simulink model "lab2"  (R2012b)
settings: Solver=ode45  StartTime=0.0  StopTime=10.0  RelTol=1e-3
undefined symbols (not defined in the file): des, gcbh
settings Model: Creator=Student  LastModifiedBy=Student

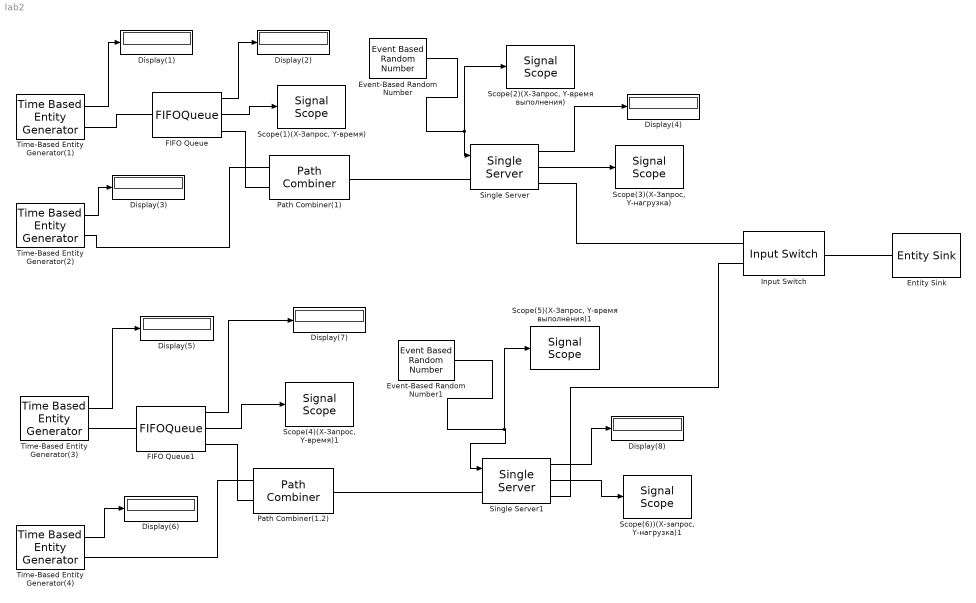
== system lab2 ==
  "Display(1) " : Display
  "Display(2) " : Display
  Display(3) : Display
  Display(4) : Display
  Display(5) : Display
  Display(6) : Display
  Display(7) : Display
  Display(8) : Display
  Entity Sink : EntitySink
  Event-Based Random Number : EventBasedRandomNumber
  Event-Based Random Number1 : EventBasedRandomNumber  meanExp=2
  FIFO Queue : FIFOQueue  StatNumberDeparted=on  StatAverageWait=on
      settings: OutputPortMap=o0,o2
  FIFO Queue1 : FIFOQueue  Capacity=30  StatNumberDeparted=on  StatAverageWait=on
      settings: OutputPortMap=o0,o2
  Input Switch : InputSwitch  NumberInputPorts=2
  Path Combiner(1) : PathCombiner  NumberInputPorts=2
  Path Combiner(1.2) : PathCombiner  NumberInputPorts=2
  "Scope(1)(X-Запрос, Y-время)" : SignalScope  LoadFcn=des.scope.CallbackSupport('seLoadFcn',gcbh)  StartFcn=des.scope.CallbackSupport('seStartFcn',gcbh)  StopFcn=des.scope.CallbackSupport('seStopFcn',gcbh)
      settings: CopyFcn=des.scope.CallbackSupport('seCopyFcn',gcbh)  DeleteFcn=des.scope.CallbackSupport('seDeleteFcn',gcbh)  PreSaveFcn=des.scope.CallbackSupport('sePreSaveFcn',gcbh)  NameChangeFcn=des.scope.CallbackSupport('seNameChangeFcn',gcbh)  OpenFcn=des.scope.CallbackSupport('seOpenFcn',gcbh)
  "Scope(2)(X-Запрос, Y-время выполнения)" : SignalScope  LoadFcn=des.scope.CallbackSupport('seLoadFcn',gcbh)  StartFcn=des.scope.CallbackSupport('seStartFcn',gcbh)  StopFcn=des.scope.CallbackSupport('seStopFcn',gcbh)
      settings: CopyFcn=des.scope.CallbackSupport('seCopyFcn',gcbh)  DeleteFcn=des.scope.CallbackSupport('seDeleteFcn',gcbh)  PreSaveFcn=des.scope.CallbackSupport('sePreSaveFcn',gcbh)  NameChangeFcn=des.scope.CallbackSupport('seNameChangeFcn',gcbh)  OpenFcn=des.scope.CallbackSupport('seOpenFcn',gcbh)
  "Scope(3)(X-Запрос, Y-нагрузка)" : SignalScope  LoadFcn=des.scope.CallbackSupport('seLoadFcn',gcbh)  StartFcn=des.scope.CallbackSupport('seStartFcn',gcbh)  StopFcn=des.scope.CallbackSupport('seStopFcn',gcbh)
      settings: CopyFcn=des.scope.CallbackSupport('seCopyFcn',gcbh)  DeleteFcn=des.scope.CallbackSupport('seDeleteFcn',gcbh)  PreSaveFcn=des.scope.CallbackSupport('sePreSaveFcn',gcbh)  NameChangeFcn=des.scope.CallbackSupport('seNameChangeFcn',gcbh)  OpenFcn=des.scope.CallbackSupport('seOpenFcn',gcbh)
  "Scope(4)(X-Запрос, Y-время)1" : SignalScope  LoadFcn=des.scope.CallbackSupport('seLoadFcn',gcbh)  StartFcn=des.scope.CallbackSupport('seStartFcn',gcbh)  StopFcn=des.scope.CallbackSupport('seStopFcn',gcbh)
      settings: CopyFcn=des.scope.CallbackSupport('seCopyFcn',gcbh)  DeleteFcn=des.scope.CallbackSupport('seDeleteFcn',gcbh)  PreSaveFcn=des.scope.CallbackSupport('sePreSaveFcn',gcbh)  NameChangeFcn=des.scope.CallbackSupport('seNameChangeFcn',gcbh)  OpenFcn=des.scope.CallbackSupport('seOpenFcn',gcbh)
  "Scope(5)(X-Запрос, Y-время выполнения)1" : SignalScope  LoadFcn=des.scope.CallbackSupport('seLoadFcn',gcbh)  StartFcn=des.scope.CallbackSupport('seStartFcn',gcbh)  StopFcn=des.scope.CallbackSupport('seStopFcn',gcbh)
      settings: CopyFcn=des.scope.CallbackSupport('seCopyFcn',gcbh)  DeleteFcn=des.scope.CallbackSupport('seDeleteFcn',gcbh)  PreSaveFcn=des.scope.CallbackSupport('sePreSaveFcn',gcbh)  NameChangeFcn=des.scope.CallbackSupport('seNameChangeFcn',gcbh)  OpenFcn=des.scope.CallbackSupport('seOpenFcn',gcbh)
  "Scope(6))(X-запрос, Y-нагрузка)1" : SignalScope  LoadFcn=des.scope.CallbackSupport('seLoadFcn',gcbh)  StartFcn=des.scope.CallbackSupport('seStartFcn',gcbh)  StopFcn=des.scope.CallbackSupport('seStopFcn',gcbh)
      settings: CopyFcn=des.scope.CallbackSupport('seCopyFcn',gcbh)  DeleteFcn=des.scope.CallbackSupport('seDeleteFcn',gcbh)  PreSaveFcn=des.scope.CallbackSupport('sePreSaveFcn',gcbh)  NameChangeFcn=des.scope.CallbackSupport('seNameChangeFcn',gcbh)  OpenFcn=des.scope.CallbackSupport('seOpenFcn',gcbh)
  Single Server : SingleServer  ServiceTimeFrom=Signal port t  PriorityServiceCompletion=50  StatNumberDeparted=on  StatUtilization=on
      settings: OutputPortMap=o0,o5
  Single Server1 : SingleServer  ServiceTimeFrom=Signal port t  PriorityServiceCompletion=50  StatNumberDeparted=on  StatUtilization=on
      settings: OutputPortMap=o0,o5
  "Time-Based Entity Generator(1) " : TimeBasedEntityGenerator  Period=3  StatNumberDeparted=on
  "Time-Based Entity Generator(2) " : TimeBasedEntityGenerator  Period=3  StatNumberDeparted=on
  Time-Based Entity Generator(3) : TimeBasedEntityGenerator  StatNumberDeparted=on
  Time-Based Entity Generator(4) : TimeBasedEntityGenerator  Period=2  StatNumberDeparted=on
  wires:
  "Time-Based Entity Generator(1) "/1 -> "Display(1) "/1
  FIFO Queue/1 -> "Display(2) "/1
  FIFO Queue/2 -> "Scope(1)(X-Запрос, Y-время)"/1
  "Time-Based Entity Generator(2) "/1 -> Display(3)/1
  Event-Based Random Number/1 -> "Scope(2)(X-Запрос, Y-время выполнения)"/1, Single Server/1
  Single Server/1 -> Display(4)/1
  Single Server/2 -> "Scope(3)(X-Запрос, Y-нагрузка)"/1
  Time-Based Entity Generator(3)/1 -> Display(5)/1
  FIFO Queue1/1 -> Display(7)/1
  FIFO Queue1/2 -> "Scope(4)(X-Запрос, Y-время)1"/1
  Time-Based Entity Generator(4)/1 -> Display(6)/1
  Event-Based Random Number1/1 -> "Scope(5)(X-Запрос, Y-время выполнения)1"/1, Single Server1/1
  Single Server1/1 -> Display(8)/1
  Single Server1/2 -> "Scope(6))(X-запрос, Y-нагрузка)1"/1
  connections:
  "Time-Based Entity Generator(1) "/RConn1 -- FIFO Queue/LConn1
  FIFO Queue/RConn1 -- Path Combiner(1)/LConn2
  "Time-Based Entity Generator(2) "/RConn1 -- Path Combiner(1)/LConn1
  Path Combiner(1)/RConn1 -- Single Server/LConn1
  Single Server/RConn1 -- Input Switch/LConn1
  Input Switch/RConn1 -- Entity Sink/LConn1
  Time-Based Entity Generator(3)/RConn1 -- FIFO Queue1/LConn1
  FIFO Queue1/RConn1 -- Path Combiner(1.2)/LConn2
  Time-Based Entity Generator(4)/RConn1 -- Path Combiner(1.2)/LConn1
  Path Combiner(1.2)/RConn1 -- Single Server1/LConn1
  Single Server1/RConn1 -- Input Switch/LConn2
